simulink model "rotpen_rl_updown"  (R2025a)
settings: Solver=VariableStepAuto  StopTime=60  AbsTol=1e-3
values from neighbouring files (symbols this model uses):
  downStart = 5    [train_updown.m]
  downVelocityScale = 10    [train_updown.m]
  dphi0 = 0    [train_updown.m]
  dtheta0 = 0    [train_updown.m]
  limitPenalty = stage2LimitPenalty    (= 100)    [train_updown.m]
  nearScale = stage2NearScale    (= 5)    [train_updown.m]
  nearWidth = 0.35    [train_updown.m]
  period = 7    [setup_updown.m]    (also in train_updown.m)
  phi0 = pi    (= 3.14159265359)    [setup_updown.m]    (also in train_updown.m)
  q1 = 1    [train_updown.m]
  q2 = 1    [train_updown.m]
  q3 = 0.01    [train_updown.m]
  q4 = 0.01    [train_updown.m]
  q5 = 2    [train_updown.m]
  q6 = 20    [train_updown.m]
  theta0 = 0    [train_updown.m]
  theta_limit = pi/2    (= 1.57079632679)    [setup_updown.m]    (also in train_updown.m)
  Ts = 0.01    [setup_updown.m]    (also in train_updown.m)
  upEnd = 4    [train_updown.m]
  upStart = 2    [train_updown.m]
  velTau = 0.05    [train_updown.m]
  volt_limit = 6    [setup_updown.m]    (also in train_updown.m)
libraries: QuanserQube x1, rllib x1, simulink x1
settings Model: SimulationMode=accelerator  Creator=The MathWorks, Inc.  LastModifiedBy=liam
settings SolverCC: AutoScaleAbsTol=off  MaxZcPerStep=1.0
settings DataIOCC: SaveOutput=off  SaveTime=off
settings DebuggingCC: UnconnectedInputMsg=warning  UnconnectedOutputMsg=warning  UnconnectedLineMsg=warning
settings ModelReferenceCC: EnableRefExpFcnMdlSchedulingChecks=on
settings RTWCC: GPUComputeCapability=3.5  DLArmComputeVersion=19.05
settings ExplorerConfigSet: SimMechanicsOpenEditorOnUpdate=off  InternalSimMechanicsExplorerSettings="<ExplorerConfiguration><canonicalview>default</canonicalview><AnimationSetting><BasePlaybackSpeed>1.0</BasePlaybackSpeed><PlaybackSpeedFactor>1.0</PlaybackSpeedFactor></AnimationSetting><TilePanel><TileInfo><Tiles Columns=\"1\" Count=\"1\" Rows=\"1\"><Column Weight=\"1\"/><Row Weight=\"1\"/><Tile Height=\"1\" Width=\"1\" X=\"0\" Y=\"0\"/></Tiles></TileInfo><SceneInfo><SceneViewer><BGColor><R>0.60000002384185791</R><G>0.60000002384185791</G><B>0.60000002384185791</B></BGColor><Camera><DoPerspective>on</DoPerspective><Position><X>0.334156231583514596</X><Y>0.107146061295956732</Y><Z>0.154419804164132285</Z></Position><Center><X>0.145480827141795971</X><Y>0.0537418892551446009</Y><Z>0.077934111254939889</Z></Center><Up><X>-0.332530024195597795</X><Y>-0.157027945704575345</Y><Z>0.929927958110882913</Z></Up><ViewLimDist>1</ViewLimDist><YLim>0.466307658154998583</YLim><XLim>0.535390274177961367</XLim></Camera></SceneViewer></SceneInfo></TilePanel><MechEditorPanel><Cameras><Camera><Id>Camera1</Id><Value><Name>Camera1</Name><NativeCamera><PositionKeyframeSet/><CenterKeyframeSet/><UpVectorKeyframeSet/></NativeCamera></Value></Camera></Cameras><GfxPanelCameraMap><MapElement CameraMLId=\"Camera1\" GfxPanelIndex=\"0\"/></GfxPanelCameraMap><VideoCreator><PlaybackSpeedRatio>1.0</PlaybackSpeedRatio><FrameRate>30</FrameRate><VideoFormat>Motion JPEG AVI</VideoFormat><FrameSize>auto</FrameSize></VideoCreator></MechEditorPanel></ExplorerConfiguration>"

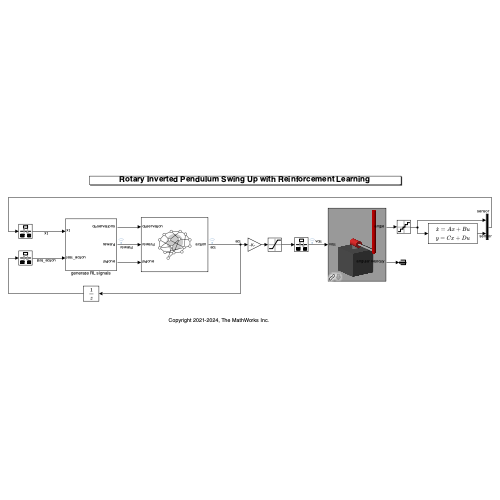
[thumbnail: Simulink's stored preview of the top-level diagram]
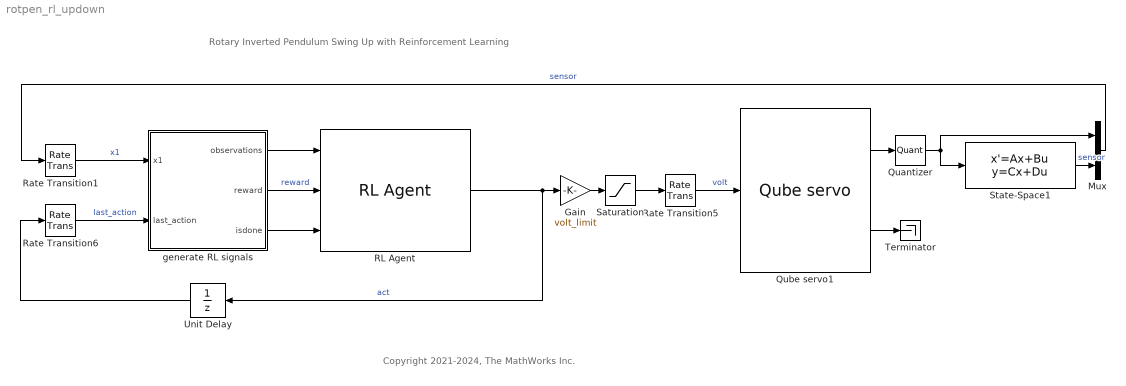
== system rotpen_rl_updown ==
  note: Rotary Inverted Pendulum Swing Up with Reinforcement Learning
  note: Copyright 2021-2024, The MathWorks Inc.
  Gain : Gain  Gain=volt_limit
  Mux : Mux  Inputs=2
  Quantizer : Quantizer  QuantizationInterval=2*pi/4096
  Qube servo1 : QuanserQube/Qube servo  a0=[theta0, phi0]  w0=[dtheta0,dphi0]  R_m=motorResistance  L_m=1.16e-3  mu_m=0.0024  K_b=0.07683  n=1  rod_mass=0.257  rod_length=0.216  rod_rad=0.01  p_mass=0.127  p_length=0.337  p_rad=0.007  D_r=dampingArm  D_p=dampingPendulum  Choice_Stopper=On
  RL Agent : rllib/RL Agent  Agent=agent  ExternalActionAsInput=off  ProvideLastAction=off  ProvideCumRwd=off  TreatAsDirectFeedthrough=on  UseStrictObservationDataTypes=off
  Rate Transition1 : RateTransition  OutPortSampleTime=Ts
  Rate Transition5 : RateTransition  OutPortSampleTime=Ts
  Rate Transition6 : RateTransition  OutPortSampleTime=Ts
  Saturation : Saturate  UpperLimit=volt_limit  LowerLimit=-volt_limit
  State-Space1 : StateSpace  A=-eye(2)/velTau  B=eye(2)/velTau  C=-eye(2)/velTau  D=eye(2)/velTau  InitialCondition=[-theta0;phi0]
  Terminator : Terminator
  Unit Delay : UnitDelay  SampleTime=-1
  generate RL signals : Subsystem
  wires:
  generate RL signals/3(isdone) -> RL Agent/3
  generate RL signals/2(reward) -> RL Agent/2  "reward"
  RL Agent/1 -> Gain/1, Unit Delay/1  "act"
  generate RL signals/1(observations) -> RL Agent/1
  Rate Transition1/1 -> generate RL signals/1(x1)  "x1"
  Unit Delay/1 -> Rate Transition6/1
  Rate Transition6/1 -> generate RL signals/2(last_action)  "last_action"
  Saturation/1 -> Rate Transition5/1
  Rate Transition5/1 -> Qube servo1/1  "volt"
  Gain/1 -> Saturation/1
  Qube servo1/1 -> Quantizer/1
  Mux/1 -> Rate Transition1/1  "sensor"
  Qube servo1/2 -> Terminator/1
  Quantizer/1 -> State-Space1/1, Mux/1
  State-Space1/1 -> Mux/2  "sensor"

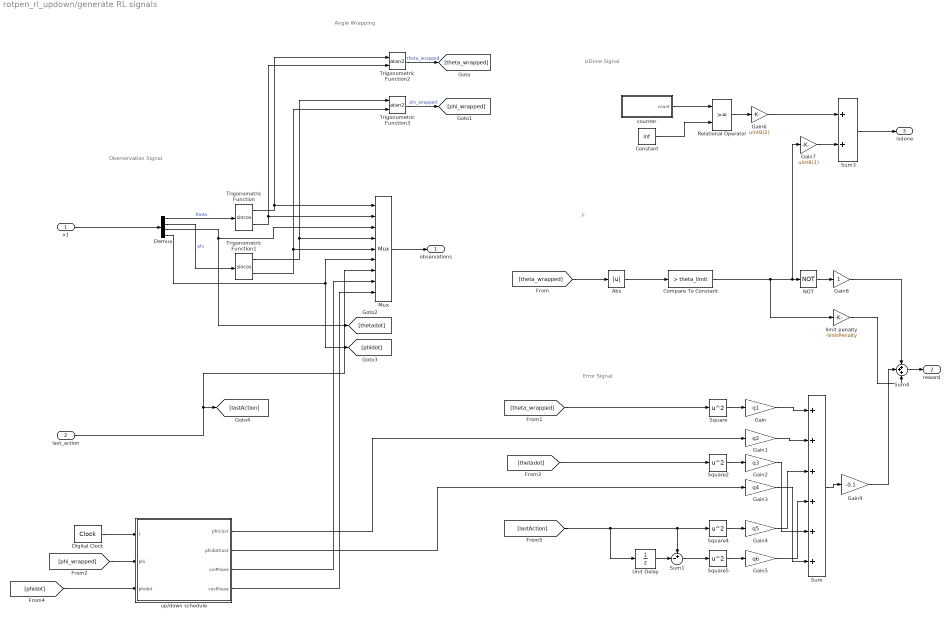
== system rotpen_rl_updown/generate RL signals ==
  note: Oberservation Signal
  note: Error Signal
  note: isDone Signal
  note: Angle Wrapping
  note: F
  x1 : Inport  SampleTime=Ts
  last_action : Inport  Port=2
  Abs : Abs  SaturateOnIntegerOverflow=off
  Compare To Constant : simulink/Logic and Bit Operations/Compare To Constant  relop=>  const=theta_limit  OutDataTypeStr=boolean
  Constant : Constant  Value=inf
  Demux : Demux
  Digital Clock : DigitalClock  SampleTime=Ts
  Gain : Gain  Gain=q1
  Gain1 : Gain  Gain=q2
  Gain2 : Gain  Gain=q3
  Gain3 : Gain  Gain=q4
  Gain4 : Gain  Gain=q5
  Gain5 : Gain  Gain=q6
  Gain6 : Gain  Gain=uint8(2)  OutDataTypeStr=uint8
  Gain7 : Gain  Gain=uint8(1)  OutDataTypeStr=uint8
  Gain8 : Gain  OutDataTypeStr=double
  Gain9 : Gain  Gain=-0.1
  Mux : Mux  Inputs=9
  NOT : Logic  Operator=NOT  IconShape=distinctive  AllPortsSameDT=off  OutDataTypeStr=boolean
  Relational Operator : RelationalOperator  OutDataTypeStr=boolean  RndMeth=Simplest  InputSameDT=off
  Square{,2,4..5} (4 alike) : Math  Operator=square
  Sum : Sum  Inputs=++++++
  Sum1 : Sum  Inputs=+-|
  Sum3 : Sum
  Sum4 : Sum  Inputs=+++
  Trigonometric Function : Trigonometry  Operator=sincos
  Trigonometric Function1 : Trigonometry  Operator=sincos
  Trigonometric Function2 : Trigonometry  Operator=atan2
  Trigonometric Function3 : Trigonometry  Operator=atan2
  Unit Delay : UnitDelay  SampleTime=-1
  counter : Subsystem
  limit penalty : Gain  Gain=-limitPenalty  OutDataTypeStr=double
  up/down schedule : MATLAB Function  TreatAsAtomicUnit=on
  observations : Outport
  reward : Outport  Port=2
  isdone : Outport  Port=3
  wires:
  Trigonometric Function1/1 -> Trigonometric Function3/1, Mux/4
  Gain9/1 -> Sum4/2
  Unit Delay/1 -> Sum1/2
  Trigonometric Function2/1 -> [theta_wrapped]  "theta_wrapped"
  Mux/1 -> observations/1
  Trigonometric Function1/2 -> Trigonometric Function3/2, Mux/5
  Square5/1 -> Gain5/1
  Gain8/1 -> Sum4/1
  Square/1 -> Gain/1
  NOT/1 -> Gain8/1
  Square4/1 -> Gain4/1
  Gain1/1 -> Sum/2
  Sum4/1 -> reward/1
  counter/1(count) -> Relational Operator/1
  Trigonometric Function/2 -> Trigonometric Function2/2, Mux/2
  x1/1 -> Demux/1
  Relational Operator/1 -> Gain6/1
  Constant/1 -> Relational Operator/2
  Sum3/1 -> isdone/1
  Trigonometric Function/1 -> Trigonometric Function2/1, Mux/1
  Sum/1 -> Gain9/1
  Sum1/1 -> Square5/1
  Abs/1 -> Compare To Constant/1
  Gain/1 -> Sum/1
  [theta_wrapped] -> Abs/1
  last_action/1 -> Mux/7, [lastAction]
  Trigonometric Function3/1 -> [phi_wrapped]  "phi_wrapped"
  [theta_wrapped] -> Square/1
  [lastAction] -> Sum1/1, Square4/1, Unit Delay/1
  Gain6/1 -> Sum3/1
  Gain7/1 -> Sum3/2
  Gain4/1 -> Sum/3
  Gain5/1 -> Sum/4
  Demux/4 -> [phidot], Mux/6
  Square2/1 -> Gain2/1
  Gain2/1 -> Sum/5
  Gain3/1 -> Sum/6
  Compare To Constant/1 -> Gain7/1, NOT/1, limit penalty/1
  Demux/1 -> Trigonometric Function/1  "theta"
  Demux/2 -> Trigonometric Function1/1  "phi"
  Demux/3 -> Mux/3, [thetadot]
  [thetadot] -> Square2/1
  Digital Clock/1 -> up/down schedule/1(t)
  [phi_wrapped] -> up/down schedule/2(phi)
  [phidot] -> up/down schedule/3(phidot)
  up/down schedule/1(phiCost) -> Gain1/1
  up/down schedule/2(phidotCost) -> Gain3/1
  up/down schedule/3(sinPhase) -> Mux/8
  up/down schedule/4(cosPhase) -> Mux/9
  limit penalty/1 -> Sum4/3

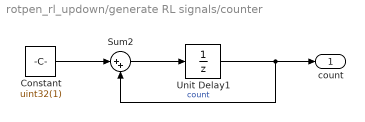
== system rotpen_rl_updown/generate RL signals/counter ==
  Constant : Constant  Value=uint32(1)
  Sum2 : Sum  Inputs=|++
  Unit Delay1 : UnitDelay  SampleTime=Ts
  count : Outport  OutDataTypeStr=uint32
  wires:
  Sum2/1 -> Unit Delay1/1
  Unit Delay1/1 -> count/1, Sum2/2  "count"
  Constant/1 -> Sum2/1

== matlab function rotpen_rl_updown/generate RL signals/up//down schedule ==
  data: t input; phiCost output; phi input; phidot input; phidotCost output; sinPhase output; cosPhase output; period parameter; upStart parameter; upEnd parameter; downStart parameter; downVelocityScale parameter; nearScale parameter; nearWidth parameter
function [phiCost, phidotCost, sinPhase, cosPhase] = schedule(t, phi, phidot, period, upStart, upEnd, downStart, downVelocityScale, nearScale, nearWidth)
% Reward schedule(repeats every period seconds): 0-2 s swing up, 2-4 s hold upright, 4-5 s fall and brake, 5-7 s hold down
% Parameters set in training script:
% - period: Length of one cycle (s)
% - upStart, upEnd: Hold upright window (s into the cycle)
% - downStart: Hold down from here to the end of the cycle (s)
% - downVelocityScale: Extra phidot penalty while holding down
% - nearScale: Size of the narrow cost around each target
% - nearWidth: Width of the narrow cost (rad)

phase = mod(t, period);
phiCost = 0;
phidotCost = phidot^2;
if phase >= upStart && phase < upEnd
    phiCost = targetCost(phi, nearScale, nearWidth);  % phi is 0 upright
elseif phase >= downStart
    phiError = atan2(sin(phi - pi), cos(phi - pi));
    phiCost = targetCost(phiError, nearScale, nearWidth);
    phidotCost = downVelocityScale * phidot^2;
end
sinPhase = sin(2*pi*phase/period);
cosPhase = cos(2*pi*phase/period);
end

function cost = targetCost(err, nearScale, nearWidth)
cost = err^2 + nearScale*(1 - exp(-(err/nearWidth)^2));
end
